simulink model "HorizontalBaseline"  (R2026b)
settings: Solver=FixedStepDiscrete  StopTime=inf  FixedStep=Official.Step
PostLoadFcn:
  | run(fullfile(fileparts(get_param('StampFly_IMU400','FileName')),'config','startup.m'));
InitFcn:
  | init_imu_flight;
undefined symbols (not defined in the file): Official
libraries: slpidlib x7, simulink x4, mspfiltlib x1
(part 5 of 5)

== stateflow chart HorizontalBaseline/OfficialFlightSupervisor ==
  settings: description=|
      | 飛行モードの状態遷移図（400 Hz）
      | INIT→AVERAGE→PARKING→FLIGHT→LANDING。通信途絶・OverG・ボタンを遷移条件で判断。
      | CycleInputsが1周期分の入力を整理し、syncで前周期の確定状態に同期、decideで今回の遷移を実行。
      | branchは今回の分岐開始状態、modeは今回の判断後の状態。MATLAB関数はChart内に置かない。
  state FlightModes [parallel]
    settings: executionOrder=1
    state PARKING
      en: mode=uint8(3);
    state AVERAGE
      en: mode=uint8(1);
    state INIT
      en: mode=uint8(0);
    state FLIGHT
      en: mode=uint8(2);
    state LANDING
      en: mode=uint8(5);
    state OTHER
      en: mode=branch;
    (default) -> INIT : /{calibration=uint16(0); buttonCounter=int8(0); buttonState=uint8(0); chatter=uint8(0); lastAHRS=uint8(0); connectionCounter=uint16(0); buttonEvent=false; calibrationDone=false;}
    AVERAGE -> PARKING : decide[calibrationDone]
    INIT -> AVERAGE : decide
    (junction 43) -> AVERAGE [order 2] : [branch==uint8(1)]
    (junction 43) -> INIT [order 1] : [branch==uint8(0)]
    PARKING -> FLIGHT : decide[buttonEvent]/{ahrsReset=true;}
    FLIGHT -> PARKING [order 1] : decide[flags(1)==1]/{ahrsReset=true;}
    (junction 43) -> PARKING [order 3] : [branch==uint8(3)]
    LANDING -> PARKING : decide[buttonEvent]
    FLIGHT -> LANDING [order 2] : decide[buttonEvent || connected==0]/{ahrsReset=true;}
    (junction 43) -> LANDING [order 5] : [branch==uint8(5)]
    (junction 43) -> FLIGHT [order 4] : [branch==uint8(2)]
    FlightModes -> (junction 43) : sync
    (junction 43) -> OTHER [order 6]
  state CycleInputs [parallel]
    en: branch=previousMode; mode=branch; ahrsReset=false; parkingReset=branch==3;
    buttonEvent=false; calibrationDone=false;
    if newPacket~=0, connectionCounter=uint16(0); end
    connected=uint8(connectionCounter<uint16(40));
    if branch==1
    calibrationDone=calibration>=uint16(800);
    if ~calibrationDone, calibration=calibration+uint16(1); end
    elseif branch~=0
    if button==1
    buttonCounter=buttonCounter+int8(1);
    if buttonCounter>int8(10),buttonCounter=int8(10);buttonState=uint8(1);end
    else
    buttonCounter=buttonCounter-int8(1);
    if buttonCounter<int8(-10),buttonCounter=int8(-10);buttonState=uint8(0);end
    end
    if chatter==0
    if buttonState==1,chatter=uint8(1);end
    elseif buttonState==0
    chatter=chatter+uint8(1);
    if chatter>uint8(40),chatter=uint8(0);buttonEvent=true;end
    end
    if branch==3
    if ahrsFlag~=lastAHRS
    if ahrsFlag==1,ahrsReset=true;end
    lastAHRS=ahrsFlag;
    end
    elseif branch==2
    connectionCounter=uint16(mod(double(connectionCounter)+1,65536));
    connected=uint8(connectionCounter<uint16(40));
    end
    end
    send(sync,FlightModes);
    send(decide,FlightModes);
    du: branch=previousMode; mode=branch; ahrsReset=false; parkingReset=branch==3;
    buttonEvent=false; calibrationDone=false;
    if newPacket~=0, connectionCounter=uint16(0); end
    connected=uint8(connectionCounter<uint16(40));
    if branch==1
    calibrationDone=calibration>=uint16(800);
    if ~calibrationDone, calibration=calibration+uint16(1); end
    elseif branch~=0
    if button==1
    buttonCounter=buttonCounter+int8(1);
    if buttonCounter>int8(10),buttonCounter=int8(10);buttonState=uint8(1);end
    else
    buttonCounter=buttonCounter-int8(1);
    if buttonCounter<int8(-10),buttonCounter=int8(-10);buttonState=uint8(0);end
    end
    if chatter==0
    if buttonState==1,chatter=uint8(1);end
    elseif buttonState==0
    chatter=chatter+uint8(1);
    if chatter>uint8(40),chatter=uint8(0);buttonEvent=true;end
    end
    if branch==3
    if ahrsFlag~=lastAHRS
    if ahrsFlag==1,ahrsReset=true;end
    lastAHRS=ahrsFlag;
    end
    elseif branch==2
    connectionCounter=uint16(mod(double(connectionCounter)+1,65536));
    connected=uint8(connectionCounter<uint16(40));
    end
    end
    send(sync,FlightModes);
    send(decide,FlightModes);
    settings: executionOrder=2
  note: 飛行モードの状態遷移図（400 Hz）
      | INIT→AVERAGE→PARKING→FLIGHT→LANDING。通信途絶・OverG・ボタンを遷移条件で判断。
      | CycleInputsが1周期分の入力を整理し、syncで前周期の確定状態に同期、decideで今回の遷移を実行。
      | branchは今回の分岐開始状態、modeは今回の判断後の状態。MATLAB関数はChart内に置かない。
  data: previousMode input uint8; button input uint8; newPacket input uint8; flags input uint8; ahrsFlag input uint8; branch output uint8; mode output uint8; ahrsReset output boolean; parkingReset output boolean; connected output uint8; calibration local uint16; buttonCounter local int8; buttonState local uint8; chatter local uint8; lastAHRS local uint8; connectionCounter local uint16; buttonEvent local boolean; calibrationDone local boolean
  events: sync local FUNCTION_CALL_EVENT; decide local FUNCTION_CALL_EVENT
